simulink model "day16_thermal_control"  (R2025b)
settings: Solver=VariableStepAuto  StartTime=0.0  StopTime=4200  RelTol=1e-3
settings Model: Creator=User  LastModifiedBy=User

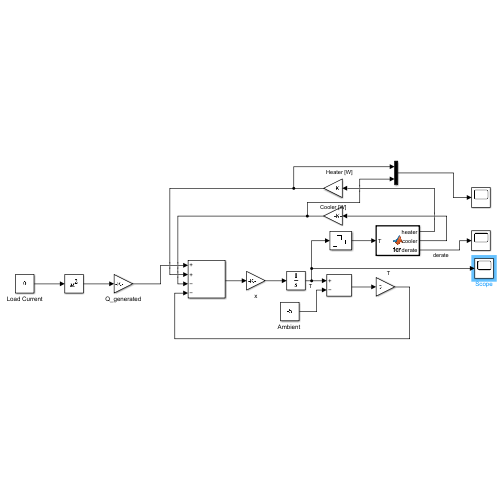
[thumbnail: Simulink's stored preview of the top-level diagram]
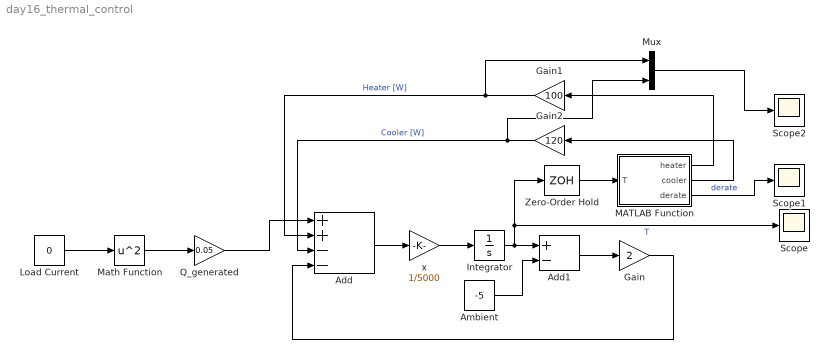
== system day16_thermal_control ==
  Add : Sum  Inputs=++--
  Add1 : Sum  Inputs=+-
  "Ambient " : Constant  Value=-5
  Gain : Gain  Gain=2
  Gain1 : Gain  Gain=100
  Gain2 : Gain  Gain=120
  Integrator : Integrator  InitialCondition=-5
  Load Current : Constant  Value=0
  MATLAB Function : MATLAB Function  TreatAsAtomicUnit=on
  Math Function : Math  Operator=square
  Mux : Mux  Inputs=2
  Q_generated : Gain  Gain=0.05
  Scope : Scope
      settings: ActiveDisplayYMinimum=-8.1257027392495722  ActiveDisplayYMaximum=23.131324653246146  YLabel=Temperature [°C]
  Scope1 : Scope
      settings: ActiveDisplayYMinimum=-0.12499999999999997  ActiveDisplayYMaximum=1.125
  Scope2 : Scope
      settings: ActiveDisplayYMinimum=-12.499999999999996  ActiveDisplayYMaximum=112.5  YLabel=Power[W]  DataLoggingVariableName=ScopeData2
  Zero-Order Hold : ZeroOrderHold
  x : Gain  Gain=1/5000
  wires:
  Load Current/1 -> Math Function/1
  Math Function/1 -> Q_generated/1
  Q_generated/1 -> Add/1
  Add/1 -> x/1
  x/1 -> Integrator/1
  Integrator/1 -> Scope/1, Zero-Order Hold/1, Add1/1  "T"
  "Ambient "/1 -> Add1/2
  Add1/1 -> Gain/1
  Gain/1 -> Add/4
  Zero-Order Hold/1 -> MATLAB Function/1(T)
  MATLAB Function/1(heater) -> Gain1/1
  Gain1/1 -> Mux/1, Add/2  "Heater [W]"
  MATLAB Function/2(cooler) -> Gain2/1
  Gain2/1 -> Mux/2, Add/3  "Cooler [W]"
  MATLAB Function/3(derate) -> Scope1/1  "derate"
  Mux/1 -> Scope2/1

== matlab function day16_thermal_control/MATLAB Function ==
  data: T input; heater output; cooler output; derate output
function [heater, cooler, derate] = fcn(T)
% T      : battery temperature [degC]
% heater : 1 = heater on      cooler : 1 = cooler on
% derate : 1 = ask the vehicle/charger to limit the current
persistent h c
if isempty(h), h = 0; c = 0; end

% heater with hysteresis: on below 15 degC, off above 20 degC
if T < 15
    h = 1;
elseif T > 20
    h = 0;
end

% cooler with hysteresis: on above 35 degC, off below 30 degC
if T > 35
    c = 1;
elseif T < 30
    c = 0;
end

% protection: outside the safe range, request a current limit
derate = double(T > 55 || T < 0);

heater = double(h);
cooler = double(c);
end
